simulink subsystem "encodervelocidad"  (R2022b)
settings: Solver=VariableStepAuto  StartTime=0.0  StopTime=10.0  RelTol=1e-3
libraries: arduinosensorlib x2
settings Model: Creator=miriamfreiriasanjuan  LastModifiedBy=miriamfreiriasanjuan

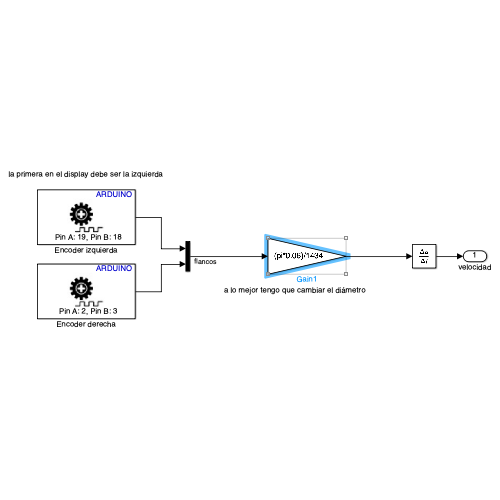
[thumbnail: Simulink's stored preview of the top-level diagram]
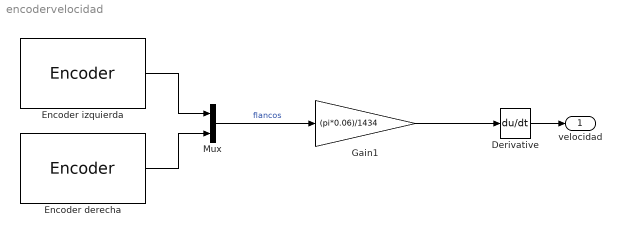
== system encodervelocidad ==
  Derivative : Derivative
  Encoder derecha : arduinosensorlib/Encoder  InputA=2  InputB=3  Mode=No reset  SampleTime=-1
  Encoder izquierda : arduinosensorlib/Encoder  InputA=19  InputB=18  Mode=No reset  SampleTime=-1
  Gain1 : Gain  Gain=(pi*0.06)/1434  OutDataTypeStr=double
  Mux : Mux  Inputs=2
  velocidad : Outport
  wires:
  Mux/1 -> Gain1/1  "flancos"
  Derivative/1 -> velocidad/1
  Gain1/1 -> Derivative/1
  Encoder izquierda/1 -> Mux/1
  Encoder derecha/1 -> Mux/2
